simulink model "Stabilizer_QDrone_048378_RollI"  (Simulink 9.3)
settings: Solver=ode2  StartTime=0.0  StopTime=inf  FixedStep=0.001  RelTol=1e-3  EnableMultiTasking=on
InitFcn:
  | addpath('D:\QDrone\QDrone_Control\pid_diagnostics');
undefined symbols (not defined in the file): Controller_, datetime, GyroCal_, HIL, m, Motors_, qc_get_step_size, QDrone_, RollI_, saved_data, Stabilizer_
libraries: quarc_library x32, simulink_extras x5, simulink x4
(part 2 of 2)

== matlab function STABILIZER - QDRONE/Bounded Roll Integral ==
  settings: updateMethod=DISCRETE  sampleTime=0.001
  data: errorRate input double size=[3 1]; term output double size=[3 1]; arm input double; throttle input double; ready input double; mode input double; angles input double size=[3 1]; gyro input double size=[3 1]; limited input double; active output double
function [term,active]=step(errorRate,arm,throttle,ready,mode,angles,gyro,limited)
%#codegen
[term,active]=qdrone_roll_i_step(errorRate,arm,throttle,ready,mode,angles,gyro,limited);
end

== matlab function PHYSICAL PLANT w// LINEAR THRUST/Red - Low Voltage Green - Armed Blue - Disarmed/MATLAB Function LED Color Assignment ==
  data: arm input double; value output double; low_battery input double
function value = fcn(arm, low_battery)

if low_battery
    value = 1;
elseif arm
    value = 2;
else 
    value = 3;
end
